simulink model "dbs_closed_loop"  (R2025a)
settings: Solver=ode4  StartTime=0.0  StopTime=Tstop  FixedStep=Tstep  RelTol=1e-3
undefined symbols (not defined in the file or in its folder): bpf_den, bpf_num, cl_enable, fhn_a, fhn_b, fhn_k, fhn_tau, fhn_v0, fhn_w0, Iext_on, Kd, Ki, Kp, Nd, ol_amp, ol_enable, pulse_gain, r_ref, rms_den, rms_num, sigma, stim_dc, stim_delayN, stim_N, stim_pwN, t_on, Tlog, Tn, Ts, Tstep, uMax
libraries: simulink x1, slpidlib x1
settings Model: Creator=apple  LastModifiedBy=apple

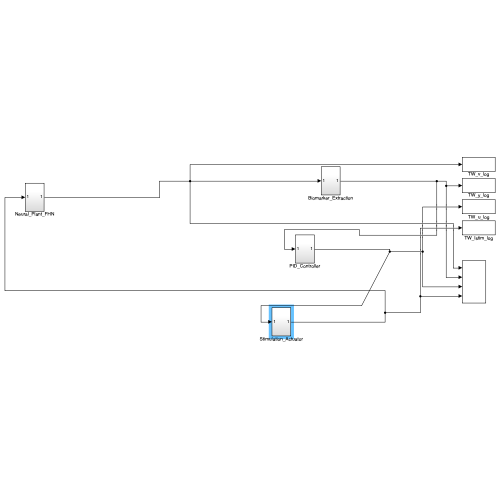
[thumbnail: Simulink's stored preview of the top-level diagram]
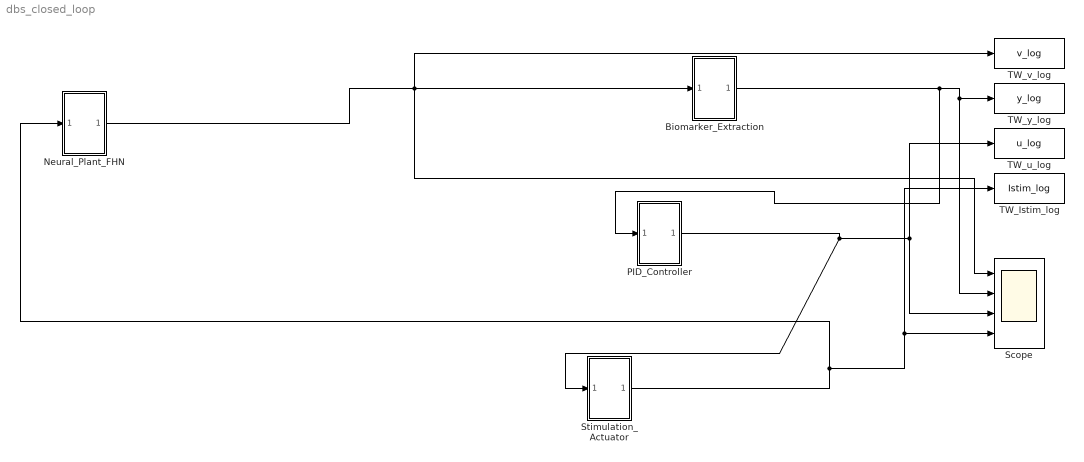
== system dbs_closed_loop ==
  Biomarker_Extraction : Subsystem
  Neural_Plant_FHN : Subsystem
  PID_Controller : Subsystem
  Scope : Scope  NumInputPorts=4
  Stimulation_Actuator : Subsystem
  TW_Istim_log : ToWorkspace  VariableName=Istim_log  SampleTime=Tlog
  TW_u_log : ToWorkspace  VariableName=u_log  SampleTime=Tlog
  TW_v_log : ToWorkspace  VariableName=v_log  SampleTime=Tlog
  TW_y_log : ToWorkspace  VariableName=y_log  SampleTime=Tlog
  wires:
  Neural_Plant_FHN/1(Out1) -> Biomarker_Extraction/1(In1), TW_v_log/1, Scope/1
  Biomarker_Extraction/1(Out1) -> PID_Controller/1(In1), TW_y_log/1, Scope/2
  PID_Controller/1(Out1) -> Stimulation_Actuator/1(In1), TW_u_log/1, Scope/3
  Stimulation_Actuator/1(Out1) -> TW_Istim_log/1, Scope/4, Neural_Plant_FHN/1(In1)

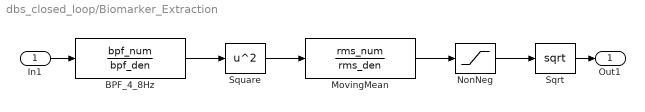
== system dbs_closed_loop/Biomarker_Extraction ==
  In1 : Inport
  BPF_4_8Hz : DiscreteTransferFcn  Numerator=bpf_num  Denominator=bpf_den  SampleTime=Ts
  MovingMean : DiscreteTransferFcn  Numerator=rms_num  Denominator=rms_den  SampleTime=Ts
  NonNeg : Saturate  UpperLimit=inf  LowerLimit=0
  Sqrt : Math  Operator=sqrt
  Square : Math  Operator=square
  Out1 : Outport
  wires:
  Sqrt/1 -> Out1/1
  Square/1 -> MovingMean/1
  In1/1 -> BPF_4_8Hz/1
  BPF_4_8Hz/1 -> Square/1
  MovingMean/1 -> NonNeg/1
  NonNeg/1 -> Sqrt/1

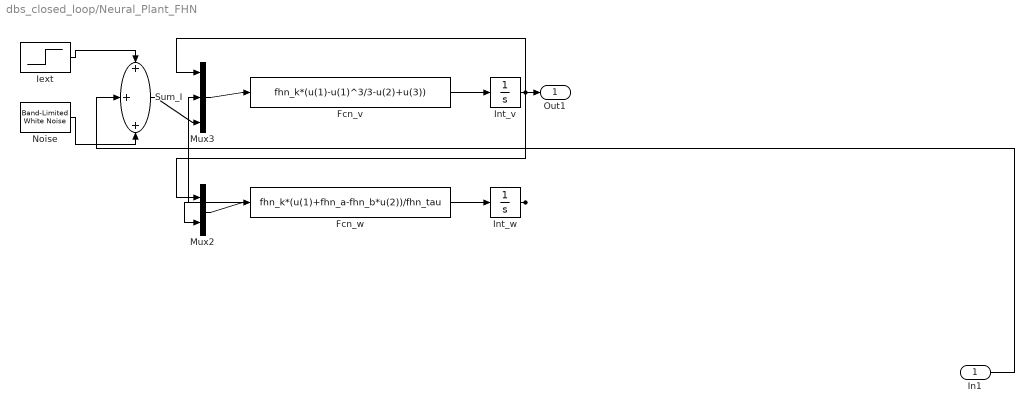
== system dbs_closed_loop/Neural_Plant_FHN ==
  In1 : Inport
  Fcn_v : Fcn  Expr=fhn_k*(u(1)-u(1)^3/3-u(2)+u(3))
  Fcn_w : Fcn  Expr=fhn_k*(u(1)+fhn_a-fhn_b*u(2))/fhn_tau
  Iext : Step  Time=t_on  After=Iext_on  SampleTime=0
  Int_v : Integrator  InitialCondition=fhn_v0
  Int_w : Integrator  InitialCondition=fhn_w0
  Mux2 : Mux  Inputs=2
  Mux3 : Mux  Inputs=3
  Noise : simulink/Sources/Band-Limited White Noise  Cov=sigma^2*Tn  Ts=Tn  seed=[23341]
  Sum_I : Sum  Inputs=+++
  Out1 : Outport
  wires:
  In1/1 -> Sum_I/2
  Mux3/1 -> Fcn_v/1
  Noise/1 -> Sum_I/3
  Sum_I/1 -> Mux3/3
  Fcn_w/1 -> Int_w/1
  Fcn_v/1 -> Int_v/1
  Int_w/1 -> Mux3/2, Mux2/2
  Iext/1 -> Sum_I/1
  Int_v/1 -> Mux3/1, Mux2/1, Out1/1
  Mux2/1 -> Fcn_w/1

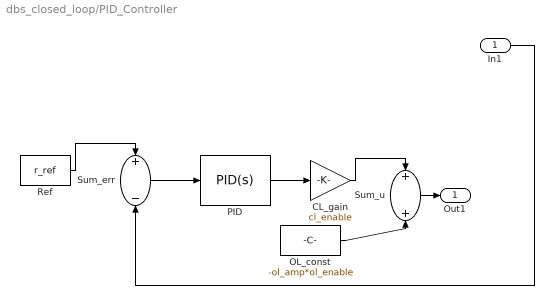
== system dbs_closed_loop/PID_Controller ==
  In1 : Inport
  CL_gain : Gain  Gain=cl_enable
  OL_const : Constant  Value=-ol_amp*ol_enable
  PID : slpidlib/PID Controller  Controller=PID  Form=Parallel  TimeDomain=Continuous-time  UseExternalTs=off  SampleTime=-1  IntegratorMethod=Forward Euler  FilterMethod=Forward Euler  ControllerParametersSource=internal  P=Kp  I=Ki  UseKiTs=off  D=Kd  UseExternalDerivativeSource=off  N=Nd  UseFilter=on  TunerSelectOption=Transfer Function Based (PID Tuner App)  InitialConditionSource=internal  InitialConditionForIntegrator=0  InitialConditionForFilter=0  DifferentiatorICPrevScaledInput=0  ExternalReset=none  TrackingMode=off  Kt=1  LimitOutput=on  SatLimitsSource=internal  UpperSaturationLimit=0  LowerSaturationLimit=-uMax  LinearizeAsGain=on  AntiWindupMode=clamping  Kb=1  LimitIntegrator=off  UpperIntegratorSaturationLimit=inf  LowerIntegratorSaturationLimit=-inf  POutMin=[]  POutMax=[]  IOutMin=[]  IOutMax=[]  DOutMin=[]  DOutMax=[]  NOutMin=[]  NOutMax=[]  SumOutMin=[]  SumOutMax=[]  SaturationOutMin=[]  SaturationOutMax=[]  PParamMin=[]  PParamMax=[]  IParamMin=[]  IParamMax=[]  DParamMin=[]  DParamMax=[]  NParamMin=[]  NParamMax=[]  KbParamMin=[]  KbParamMax=[]  KtParamMin=[]  KtParamMax=[]  KbOutMin=[]  KbOutMax=[]  KtOutMin=[]  KtOutMax=[]  IntegratorOutMin=[]  IntegratorOutMax=[]  FilterOutMin=[]  FilterOutMax=[]  SumI1OutMin=[]  SumI1OutMax=[]  SumI2OutMin=[]  SumI2OutMax=[]  SumI3OutMin=[]  SumI3OutMax=[]  SumI4OutMin=[]  SumI4OutMax=[]  SumDOutMin=[]  SumDOutMax=[]  DifferentiatorOutMin=[]  DifferentiatorOutMax=[]  FilterDiffOutCoefMin=[]  FilterDiffOutCoefMax=[]  ReciprocalOutMin=[]  ReciprocalOutMax=[]  SumDenOutMin=[]  SumDenOutMax=[]  SumNumOutMin=[]  SumNumOutMax=[]  DivideOutMin=[]  DivideOutMax=[]  UdiffTsProdOutMin=[]  UdiffTsProdOutMax=[]  NTsProdOutMin=[]  NTsProdOutMax=[]  UintegralTsProdOutMin=[]  UintegralTsProdOutMax=[]  UngainTsProdOutMin=[]  UngainTsProdOutMax=[]  ClampingZeroOutDataTypeStr=Inherit: Inherit via back propagation  ClampingZeroOutMin=[]  ClampingZeroOutMax=[]  FilterDenConstantOutDataTypeStr=Inherit: Inherit via back propagation  FilterDenConstantOutMin=[]  FilterDenConstantOutMax=[]  PCopyOutDataTypeStr=Inherit: Inherit via back propagation  PCopyOutMin=[]  PCopyOutMax=[]  NCopyOutDataTypeStr=Inherit: Inherit via back propagation  NCopyOutMin=[]  NCopyOutMax=[]  IntegratorContinuousStateAttributes=''  IntegratorStateMustResolveToSignalObject=off  IntegratorRTWStateStorageClass=Auto  FilterContinuousStateAttributes=''  FilterStateMustResolveToSignalObject=off  FilterRTWStateStorageClass=Auto  ParallelPVariant=InternalParameters  IdealPVariant=Disabled  IVariant=InternalParameters  DVariant=InternalParameters  IntegratorVariant=Continuous  SatVariant=Enabled  AWVariant=ContClampingParallel  PCopyVariant=Disabled  TRVariant=Disabled  FdbkBlocksVariant=Forward  IdealPFdbkVariant=Disabled  SatFdbkVariant=Disabled  DerivativeFilterVariant=ContFilter  NVariant=InternalParameters  NCopyVariant=Disabled  FilterICVariant=InternalICsFilter  IntegratorICVariant=InternalICs  ExternalResetVariant=Disabled  TRSumVariant=Passthrough  SumFdbkVariant=Disabled  SumVariant=Sum_PID  TsampFilterVariant=InternalTs  TsampNgainVariant=Passthrough  TsampIntegralVariant=Disabled_SignalSpec  ExternalSaturationOutDataTypeStr=Inherit: Same as second input  DerivativeSourceVariant=ErrorSignal  PreIntVariant=InternalPreInt
  Ref : Constant  Value=r_ref
  Sum_err : Sum  Inputs=+-
  Sum_u : Sum
  Out1 : Outport
  wires:
  In1/1 -> Sum_err/2
  PID/1 -> CL_gain/1
  Sum_u/1 -> Out1/1
  CL_gain/1 -> Sum_u/1
  Sum_err/1 -> PID/1
  OL_const/1 -> Sum_u/2
  Ref/1 -> Sum_err/1

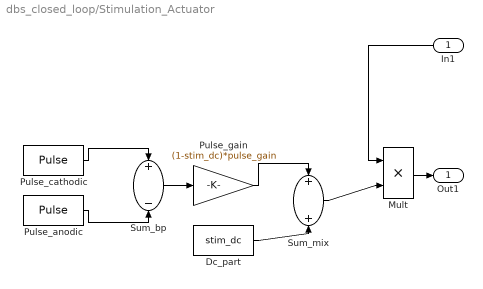
== system dbs_closed_loop/Stimulation_Actuator ==
  In1 : Inport
  Dc_part : Constant  Value=stim_dc
  Mult : Product
  Pulse_anodic : DiscretePulseGenerator  Period=stim_N  PulseWidth=stim_pwN  PhaseDelay=stim_delayN  SampleTime=Tstep
  Pulse_cathodic : DiscretePulseGenerator  Period=stim_N  PulseWidth=stim_pwN  SampleTime=Tstep
  Pulse_gain : Gain  Gain=(1-stim_dc)*pulse_gain
  Sum_bp : Sum  Inputs=+-
  Sum_mix : Sum
  Out1 : Outport
  wires:
  In1/1 -> Mult/1
  Sum_mix/1 -> Mult/2
  Dc_part/1 -> Sum_mix/2
  Pulse_anodic/1 -> Sum_bp/2
  Mult/1 -> Out1/1
  Sum_bp/1 -> Pulse_gain/1
  Pulse_gain/1 -> Sum_mix/1
  Pulse_cathodic/1 -> Sum_bp/1
